simulink model "simu1"  (R2025b)
settings: Solver=VariableStepAuto  StartTime=0.0  StopTime=10.0  RelTol=1e-3
settings Model: Creator=ThinkPad  LastModifiedBy=ThinkPad

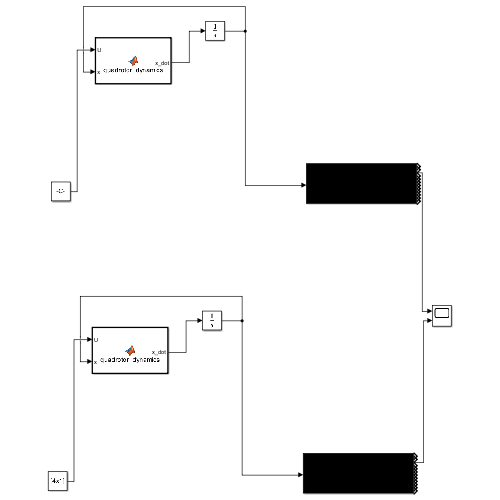
[thumbnail: Simulink's stored preview of the top-level diagram]
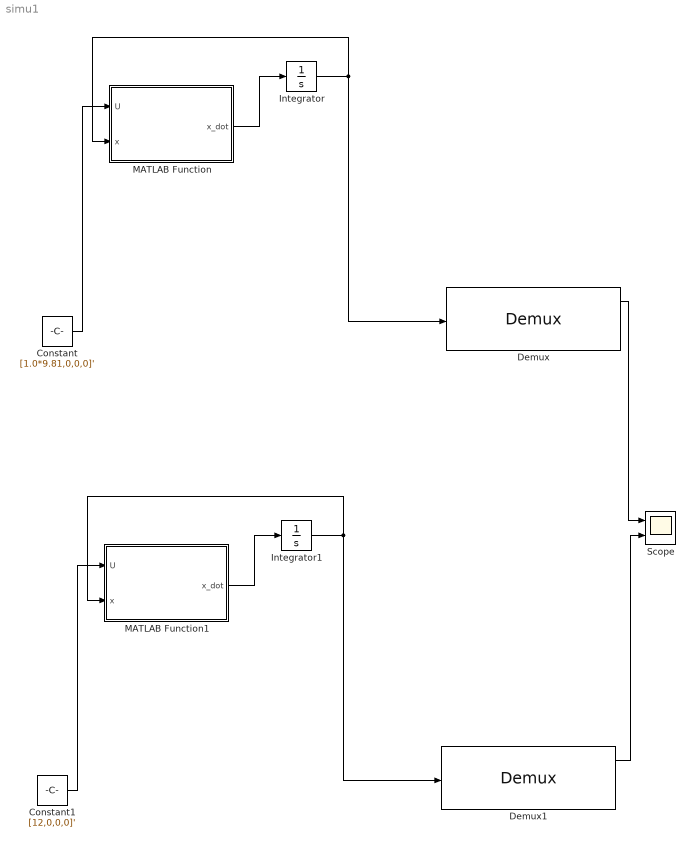
== system simu1 ==
  Constant : Constant  Value=[1.0*9.81,0,0,0]'
  Constant1 : Constant  Value=[12,0,0,0]'
  Demux : Demux  Outputs=12
  Demux1 : Demux  Outputs=12
  Integrator : Integrator  InitialCondition=zeros(12,1)
  Integrator1 : Integrator  InitialCondition=zeros(12,1)
  MATLAB Function : MATLAB Function  TreatAsAtomicUnit=on
  MATLAB Function1 : MATLAB Function  TreatAsAtomicUnit=on
  Scope : Scope  NumInputPorts=2
      settings: ActiveDisplayYMinimum=-13.6875  ActiveDisplayYMaximum=123.18750000000003  DataLoggingVariableName=Figure_Simu_1
  wires:
  MATLAB Function/1(x_dot) -> Integrator/1
  Integrator/1 -> Demux/1, MATLAB Function/2(x)
  Constant/1 -> MATLAB Function/1(U)
  Constant1/1 -> MATLAB Function1/1(U)
  Integrator1/1 -> Demux1/1, MATLAB Function1/2(x)
  MATLAB Function1/1(x_dot) -> Integrator1/1
  Demux/3 -> Scope/1
  Demux1/3 -> Scope/2

== matlab function simu1/MATLAB Function ==
  data: U input; x_dot output; x input
function x_dot = quadrotor_dynamics(U, x)
    % 1. Thông số vật lý
    m = 1.0; 
    g = 9.81;
    Ix = 0.008;
    Iy = 0.008;
    Iz = 0.015;
    
    % 2. Tín hiệu đầu vào
    U1 = U(1);
    U2 = U(2);
    U3 = U(3);
    U4 = U(4);
    
    % 3. Trích xuất trạng thái hiện tại
    phi   = x(4);
    theta = x(5);
    psi   = x(6);
    
    v_X = x(7);  
    v_Y = x(8);
    v_Z = x(9);
    
    p = x(10);
    q = x(11);
    r = x(12);
    
    % 4. KHỞI TẠO VECTƠ (Bắt buộc phải có dòng này để hết lỗi)
    x_dot = zeros(12, 1);
    
    % 5. Phương trình động lực học
    x_dot(1) = v_X;
    x_dot(2) = v_Y;
    x_dot(3) = v_Z;
    
    x_dot(4) = p;
    x_dot(5) = q;
    x_dot(6) = r;
    
    x_dot(7) = (cos(phi)*sin(theta)*cos(psi) + sin(phi)*sin(psi)) * (U1/m);
    x_dot(8) = (cos(phi)*sin(theta)*sin(psi) - sin(phi)*cos(psi)) * (U1/m);
    x_dot(9) = -g + (cos(phi)*cos(theta)) * (U1/m);
    
    x_dot(10) = ((Iy - Iz)/Ix) * q * r + (U2/Ix);
    x_dot(11) = ((Iz - Ix)/Iy) * p * r + (U3/Iy);
    x_dot(12) = ((Ix - Iy)/Iz) * p * q + (U4/Iz);
end

== matlab function simu1/MATLAB Function1 ==
  data: U input; x_dot output; x input
function x_dot = quadrotor_dynamics(U, x)
    % 1. Thông số vật lý
    m = 1.0; 
    g = 9.81;
    Ix = 0.008;
    Iy = 0.008;
    Iz = 0.015;
    
    % 2. Tín hiệu đầu vào
    U1 = U(1);
    U2 = U(2);
    U3 = U(3);
    U4 = U(4);
    
    % 3. Trích xuất trạng thái hiện tại
    phi   = x(4);
    theta = x(5);
    psi   = x(6);
    
    v_X = x(7);  
    v_Y = x(8);
    v_Z = x(9);
    
    p = x(10);
    q = x(11);
    r = x(12);
    
    % 4. KHỞI TẠO VECTƠ (Bắt buộc phải có dòng này để hết lỗi)
    x_dot = zeros(12, 1);
    
    % 5. Phương trình động lực học
    x_dot(1) = v_X;
    x_dot(2) = v_Y;
    x_dot(3) = v_Z;
    
    x_dot(4) = p;
    x_dot(5) = q;
    x_dot(6) = r;
    
    x_dot(7) = (cos(phi)*sin(theta)*cos(psi) + sin(phi)*sin(psi)) * (U1/m);
    x_dot(8) = (cos(phi)*sin(theta)*sin(psi) - sin(phi)*cos(psi)) * (U1/m);
    x_dot(9) = -g + (cos(phi)*cos(theta)) * (U1/m);
    
    x_dot(10) = ((Iy - Iz)/Ix) * q * r + (U2/Ix);
    x_dot(11) = ((Iz - Ix)/Iy) * p * r + (U3/Iy);
    x_dot(12) = ((Ix - Iy)/Iz) * p * q + (U4/Iz);
end
